simulink model "task2_simulink"  (R2026a)
settings: Solver=VariableStepAuto  StopTime=2
settings Model: Creator=DELL  LastModifiedBy=DELL

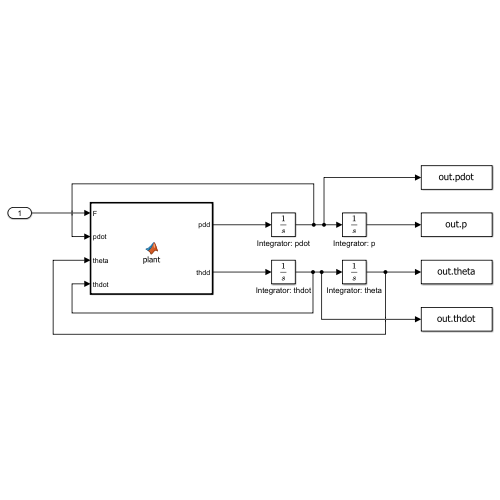
[thumbnail: Simulink's stored preview of the top-level diagram]
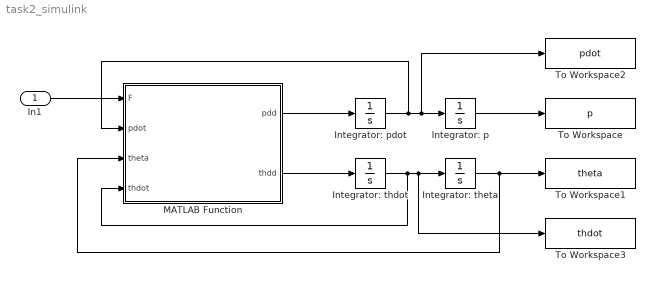
== system task2_simulink ==
  In1 : Inport
  Integrator: p : Integrator
  Integrator: pdot : Integrator
  Integrator: thdot : Integrator
  Integrator: theta : Integrator
  MATLAB Function : MATLAB Function  TreatAsAtomicUnit=on
  To Workspace : ToWorkspace  VariableName=p  SaveFormat=Timeseries  SampleTime=0.01
  To Workspace1 : ToWorkspace  VariableName=theta  SaveFormat=Timeseries  SampleTime=0.01
  To Workspace2 : ToWorkspace  VariableName=pdot  SaveFormat=Timeseries  SampleTime=-1
  To Workspace3 : ToWorkspace  VariableName=thdot  SaveFormat=Timeseries  SampleTime=-1
  wires:
  MATLAB Function/1(pdd) -> Integrator: pdot/1
  MATLAB Function/2(thdd) -> Integrator: thdot/1
  Integrator: pdot/1 -> MATLAB Function/2(pdot), To Workspace2/1, Integrator: p/1
  Integrator: thdot/1 -> MATLAB Function/4(thdot), To Workspace3/1, Integrator: theta/1
  Integrator: theta/1 -> To Workspace1/1, MATLAB Function/3(theta)
  In1/1 -> MATLAB Function/1(F)
  Integrator: p/1 -> To Workspace/1

== matlab function task2_simulink/MATLAB Function ==
  data: F input; pdd output; pdot input; theta input; thdot input; thdd output
function [pdd, thdd] = plant(F, pdot, theta, thdot)

M = 5;
m = 1;
l = 0.5;
c = 0.2;
g = 9.8;

pdd = ( ...
    F ...
    - c*pdot ...
    + m*g*sin(theta)*cos(theta) ...
    - m*l*sin(theta)*thdot^2 ...
    ) / (M+m-m*cos(theta)^2);

thdd = ( ...
    cos(theta)*pdd ...
    + g*sin(theta) ...
    ) / l;

end
